simulink model "r2_b8a4x1kf"  (R2012b)
settings: Solver=VariableStepDiscrete  SolverMode=SingleTasking  StartTime=0.0  StopTime=1  RelTol=1e-3
undefined symbols (not defined in the file): fft_stages, n_bits_ants, n_bits_xengs
libraries: xbsIndex_r4 x22142, casper_library_misc x166, xbsReplacements_r4 x24, casper_library_delays x8, xps_library x5, casper_library_communications x4
(part 7 of 178)

== system r2_b8a4x1kf/bus_expand8 ==
  bus_in : Inport
  reinterpret1 : xbsIndex_r4/Reinterpret  force_arith_type=on  arith_type=Unsigned  force_bin_pt=on  bin_pt=0  block_type=reinterpret
  reinterpret2 : xbsIndex_r4/Reinterpret  force_arith_type=on  arith_type=Unsigned  force_bin_pt=on  bin_pt=0  block_type=reinterpret
  slice1 : xbsIndex_r4/Slice  nbits=16  boolean_output=off  mode=Upper Bit Location + Width  bit1=-16  base1=MSB of Input  bit0=0  base0=LSB of Input  dbl_ovrd=off  block_type=slice
  slice2 : xbsIndex_r4/Slice  nbits=16  boolean_output=off  mode=Upper Bit Location + Width  bit1=0  base1=MSB of Input  bit0=0  base0=LSB of Input  dbl_ovrd=off  block_type=slice
  msb_out2 : Outport
  lsb_out1 : Outport  Port=2
  wires:
  bus_in/1 -> slice2/1, slice1/1
  slice2/1 -> reinterpret2/1
  reinterpret2/1 -> msb_out2/1
  slice1/1 -> reinterpret1/1
  reinterpret1/1 -> lsb_out1/1

== system r2_b8a4x1kf/bus_expand9 ==
  bus_in : Inport
  slice1 : xbsIndex_r4/Slice  nbits=1  boolean_output=on  mode=Upper Bit Location + Width  bit1=-4  base1=MSB of Input  bit0=0  base0=LSB of Input  dbl_ovrd=off  block_type=slice
  slice2 : xbsIndex_r4/Slice  nbits=1  boolean_output=on  mode=Upper Bit Location + Width  bit1=-3  base1=MSB of Input  bit0=0  base0=LSB of Input  dbl_ovrd=off  block_type=slice
  slice3 : xbsIndex_r4/Slice  nbits=1  boolean_output=on  mode=Upper Bit Location + Width  bit1=-2  base1=MSB of Input  bit0=0  base0=LSB of Input  dbl_ovrd=off  block_type=slice
  slice4 : xbsIndex_r4/Slice  nbits=1  boolean_output=on  mode=Upper Bit Location + Width  bit1=-1  base1=MSB of Input  bit0=0  base0=LSB of Input  dbl_ovrd=off  block_type=slice
  slice5 : xbsIndex_r4/Slice  nbits=1  boolean_output=on  mode=Upper Bit Location + Width  bit1=0  base1=MSB of Input  bit0=0  base0=LSB of Input  dbl_ovrd=off  block_type=slice
  msb_out5 : Outport
  out4 : Outport  Port=2
  out3 : Outport  Port=3
  out2 : Outport  Port=4
  lsb_out1 : Outport  Port=5
  wires:
  bus_in/1 -> slice5/1, slice4/1, slice3/1, slice2/1, slice1/1
  slice5/1 -> msb_out5/1
  slice4/1 -> out4/1
  slice3/1 -> out3/1
  slice2/1 -> out2/1
  slice1/1 -> lsb_out1/1

== system r2_b8a4x1kf/control ==
  convert1_{1..8,10} (9 alike) : DataTypeConversion  OutDataTypeStr=fixdt('ufix1_En0')  LockScale=on
  convert1_9 : DataTypeConversion  OutDataTypeStr=fixdt('ufix2_En0')  LockScale=on
  convert2_{1..8,10} (9 alike) : DataTypeConversion  OutDataTypeStr=fixdt('ufix1_En0')  ConvertRealWorld=Stored Integer (SI)  LockScale=on
  convert2_9 : DataTypeConversion  OutDataTypeStr=fixdt('ufix2_En0')  ConvertRealWorld=Stored Integer (SI)  LockScale=on
  gain_1 : Gain  Gain=1024
  gain_10 : Gain
  gain_2 : Gain  Gain=512
  gain_3 : Gain  Gain=256
  gain_4 : Gain  Gain=128
  gain_5 : Gain  Gain=64
  gain_6 : Gain  Gain=32
  gain_7 : Gain  Gain=16
  gain_8 : Gain  Gain=8
  gain_9 : Gain  Gain=2
  io_delay : xbsIndex_r4/Delay  rst=off  infoeditControl=Selection of Reset will increase slice count due to use of real FFs and instead of SRLs  en=off  latency=0  dbl_ovrd=off  reg_retiming=on  block_type=delay
  r2_b8a4x1kf_new_control_user_data_out : xbsIndex_r4/Gateway In  gui_display_data_type=Fixed-point  arith_type=Unsigned  n_bits=32  bin_pt=0  preci_type=Single  exp_width=8  frac_width=24  quantization="Round  (unbiased: +/- Inf)"  overflow=Saturate  period=1  dbl_ovrd=off  timing_constraint=None  locs_specified=off  LOCs={}  UseAsADC=off  ADCChannel='1'  inherit_from_input=off  hdl_port=on  block_type=gatewayin
  reint9 : xbsIndex_r4/Reinterpret  force_arith_type=on  arith_type=Unsigned  force_bin_pt=on  bin_pt=0  block_type=reinterpret
  sim_{1..10} (10 alike) : Constant  Value=0
  sim_add : Sum  Inputs=++++++++++  OutDataTypeStr=uint32
  slice_cnt_rst : xbsIndex_r4/Slice  nbits=1  boolean_output=on  mode=Lower Bit Location + Width  bit1=0  base1=MSB of Input  bit0=8  base0=LSB of Input  dbl_ovrd=off  block_type=slice
  slice_flasher_en : xbsIndex_r4/Slice  nbits=1  boolean_output=on  mode=Lower Bit Location + Width  bit1=0  base1=MSB of Input  bit0=4  base0=LSB of Input  dbl_ovrd=off  block_type=slice
  slice_gbe_debug_rst : xbsIndex_r4/Slice  nbits=1  boolean_output=on  mode=Lower Bit Location + Width  bit1=0  base1=MSB of Input  bit0=5  base0=LSB of Input  dbl_ovrd=off  block_type=slice
  slice_gbe_rst : xbsIndex_r4/Slice  nbits=1  boolean_output=on  mode=Lower Bit Location + Width  bit1=0  base1=MSB of Input  bit0=7  base0=LSB of Input  dbl_ovrd=off  block_type=slice
  slice_gbe_txen : xbsIndex_r4/Slice  nbits=1  boolean_output=on  mode=Lower Bit Location + Width  bit1=0  base1=MSB of Input  bit0=6  base0=LSB of Input  dbl_ovrd=off  block_type=slice
  slice_reord_snaptrig : xbsIndex_r4/Slice  nbits=1  boolean_output=on  mode=Lower Bit Location + Width  bit1=0  base1=MSB of Input  bit0=3  base0=LSB of Input  dbl_ovrd=off  block_type=slice
  slice_reord_snaptrigsel : xbsIndex_r4/Slice  nbits=2  boolean_output=off  mode=Lower Bit Location + Width  bit1=0  base1=MSB of Input  bit0=1  base0=LSB of Input  dbl_ovrd=off  block_type=slice
  slice_status_clr : xbsIndex_r4/Slice  nbits=1  boolean_output=on  mode=Lower Bit Location + Width  bit1=0  base1=MSB of Input  bit0=9  base0=LSB of Input  dbl_ovrd=off  block_type=slice
  slice_unpack_snapwesel : xbsIndex_r4/Slice  nbits=1  boolean_output=on  mode=Lower Bit Location + Width  bit1=0  base1=MSB of Input  bit0=0  base0=LSB of Input  dbl_ovrd=off  block_type=slice
  slice_vacc_rst : xbsIndex_r4/Slice  nbits=1  boolean_output=on  mode=Lower Bit Location + Width  bit1=0  base1=MSB of Input  bit0=10  base0=LSB of Input  dbl_ovrd=off  block_type=slice
  in_vacc_rst : Outport
  in_status_clr : Outport  Port=2
  in_cnt_rst : Outport  Port=3
  in_gbe_rst : Outport  Port=4
  in_gbe_txen : Outport  Port=5
  in_gbe_debug_rst : Outport  Port=6
  in_flasher_en : Outport  Port=7
  in_reord_snaptrig : Outport  Port=8
  in_reord_snaptrigsel : Outport  Port=9
  in_unpack_snapwesel : Outport  Port=10
  wires:
  r2_b8a4x1kf_new_control_user_data_out/1 -> io_delay/1
  sim_add/1 -> r2_b8a4x1kf_new_control_user_data_out/1
  sim_1/1 -> convert1_1/1
  convert1_1/1 -> convert2_1/1
  convert2_1/1 -> gain_1/1
  gain_1/1 -> sim_add/1
  io_delay/1 -> slice_vacc_rst/1, slice_status_clr/1, slice_cnt_rst/1, slice_gbe_rst/1, slice_gbe_txen/1, slice_gbe_debug_rst/1, slice_flasher_en/1, slice_reord_snaptrig/1, slice_reord_snaptrigsel/1, slice_unpack_snapwesel/1
  slice_vacc_rst/1 -> in_vacc_rst/1
  sim_2/1 -> convert1_2/1
  convert1_2/1 -> convert2_2/1
  convert2_2/1 -> gain_2/1
  gain_2/1 -> sim_add/2
  slice_status_clr/1 -> in_status_clr/1
  sim_3/1 -> convert1_3/1
  convert1_3/1 -> convert2_3/1
  convert2_3/1 -> gain_3/1
  gain_3/1 -> sim_add/3
  slice_cnt_rst/1 -> in_cnt_rst/1
  sim_4/1 -> convert1_4/1
  convert1_4/1 -> convert2_4/1
  convert2_4/1 -> gain_4/1
  gain_4/1 -> sim_add/4
  slice_gbe_rst/1 -> in_gbe_rst/1
  sim_5/1 -> convert1_5/1
  convert1_5/1 -> convert2_5/1
  convert2_5/1 -> gain_5/1
  gain_5/1 -> sim_add/5
  slice_gbe_txen/1 -> in_gbe_txen/1
  sim_6/1 -> convert1_6/1
  convert1_6/1 -> convert2_6/1
  convert2_6/1 -> gain_6/1
  gain_6/1 -> sim_add/6
  slice_gbe_debug_rst/1 -> in_gbe_debug_rst/1
  sim_7/1 -> convert1_7/1
  convert1_7/1 -> convert2_7/1
  convert2_7/1 -> gain_7/1
  gain_7/1 -> sim_add/7
  slice_flasher_en/1 -> in_flasher_en/1
  sim_8/1 -> convert1_8/1
  convert1_8/1 -> convert2_8/1
  convert2_8/1 -> gain_8/1
  gain_8/1 -> sim_add/8
  slice_reord_snaptrig/1 -> in_reord_snaptrig/1
  sim_9/1 -> convert1_9/1
  convert1_9/1 -> convert2_9/1
  convert2_9/1 -> gain_9/1
  gain_9/1 -> sim_add/9
  slice_reord_snaptrigsel/1 -> reint9/1
  reint9/1 -> in_reord_snaptrigsel/1
  sim_10/1 -> convert1_10/1
  convert1_10/1 -> convert2_10/1
  convert2_10/1 -> gain_10/1
  gain_10/1 -> sim_add/10
  slice_unpack_snapwesel/1 -> in_unpack_snapwesel/1

== system r2_b8a4x1kf/dest_err_cnt0 ==
  out_reg : Inport
  assert_reg : xbsIndex_r4/Assert  assert_type=on  type_source=Explicitly  gui_display_data_type=Fixed-point  arith_type=Unsigned  n_bits=16  bin_pt=0  preci_type=Single  exp_width=8  frac_width=24  assert_rate=off  rate_source=Explicitly  period=1  output_port=on  block_type=assert
  cast_gw : xbsIndex_r4/Convert  gui_display_data_type=Fixed-point  arith_type=Unsigned  n_bits=32  bin_pt=0  float_type=Single  exp_bits=8  fraction_bits=24  quantization=Truncate  overflow=Wrap  en=off  latency=0  dbl_ovrd=off  pipeline=off  block_type=convert
  io_delay : xbsIndex_r4/Delay  rst=off  infoeditControl=Selection of Reset will increase slice count due to use of real FFs and instead of SRLs  en=off  latency=0  dbl_ovrd=off  reg_retiming=on  block_type=delay
  r2_b8a4x1kf_new_dest_err_cnt0_user_data_in : xbsIndex_r4/Gateway Out  inherit_from_input=off  hdl_port=on  timing_constraint=None  locs_specified=off  LOCs={}  UseAsDAC=off  DACChannel='1'  block_type=gatewayout
  reint1 : xbsIndex_r4/Reinterpret  force_arith_type=on  arith_type=Unsigned  force_bin_pt=on  bin_pt=0  block_type=reinterpret
  sim_out : Terminator
  wires:
  io_delay/1 -> cast_gw/1
  cast_gw/1 -> r2_b8a4x1kf_new_dest_err_cnt0_user_data_in/1
  r2_b8a4x1kf_new_dest_err_cnt0_user_data_in/1 -> sim_out/1
  out_reg/1 -> assert_reg/1
  assert_reg/1 -> reint1/1
  reint1/1 -> io_delay/1

== system r2_b8a4x1kf/dest_err_cnt1 ==
  out_reg : Inport
  assert_reg : xbsIndex_r4/Assert  assert_type=on  type_source=Explicitly  gui_display_data_type=Fixed-point  arith_type=Unsigned  n_bits=16  bin_pt=0  preci_type=Single  exp_width=8  frac_width=24  assert_rate=off  rate_source=Explicitly  period=1  output_port=on  block_type=assert
  cast_gw : xbsIndex_r4/Convert  gui_display_data_type=Fixed-point  arith_type=Unsigned  n_bits=32  bin_pt=0  float_type=Single  exp_bits=8  fraction_bits=24  quantization=Truncate  overflow=Wrap  en=off  latency=0  dbl_ovrd=off  pipeline=off  block_type=convert
  io_delay : xbsIndex_r4/Delay  rst=off  infoeditControl=Selection of Reset will increase slice count due to use of real FFs and instead of SRLs  en=off  latency=0  dbl_ovrd=off  reg_retiming=on  block_type=delay
  r2_b8a4x1kf_new_dest_err_cnt1_user_data_in : xbsIndex_r4/Gateway Out  inherit_from_input=off  hdl_port=on  timing_constraint=None  locs_specified=off  LOCs={}  UseAsDAC=off  DACChannel='1'  block_type=gatewayout
  reint1 : xbsIndex_r4/Reinterpret  force_arith_type=on  arith_type=Unsigned  force_bin_pt=on  bin_pt=0  block_type=reinterpret
  sim_out : Terminator
  wires:
  io_delay/1 -> cast_gw/1
  cast_gw/1 -> r2_b8a4x1kf_new_dest_err_cnt1_user_data_in/1
  r2_b8a4x1kf_new_dest_err_cnt1_user_data_in/1 -> sim_out/1
  out_reg/1 -> assert_reg/1
  assert_reg/1 -> reint1/1
  reint1/1 -> io_delay/1

== system r2_b8a4x1kf/dest_err_cnt2 ==
  out_reg : Inport
  assert_reg : xbsIndex_r4/Assert  assert_type=on  type_source=Explicitly  gui_display_data_type=Fixed-point  arith_type=Unsigned  n_bits=16  bin_pt=0  preci_type=Single  exp_width=8  frac_width=24  assert_rate=off  rate_source=Explicitly  period=1  output_port=on  block_type=assert
  cast_gw : xbsIndex_r4/Convert  gui_display_data_type=Fixed-point  arith_type=Unsigned  n_bits=32  bin_pt=0  float_type=Single  exp_bits=8  fraction_bits=24  quantization=Truncate  overflow=Wrap  en=off  latency=0  dbl_ovrd=off  pipeline=off  block_type=convert
  io_delay : xbsIndex_r4/Delay  rst=off  infoeditControl=Selection of Reset will increase slice count due to use of real FFs and instead of SRLs  en=off  latency=0  dbl_ovrd=off  reg_retiming=on  block_type=delay
  r2_b8a4x1kf_new_dest_err_cnt2_user_data_in : xbsIndex_r4/Gateway Out  inherit_from_input=off  hdl_port=on  timing_constraint=None  locs_specified=off  LOCs={}  UseAsDAC=off  DACChannel='1'  block_type=gatewayout
  reint1 : xbsIndex_r4/Reinterpret  force_arith_type=on  arith_type=Unsigned  force_bin_pt=on  bin_pt=0  block_type=reinterpret
  sim_out : Terminator
  wires:
  io_delay/1 -> cast_gw/1
  cast_gw/1 -> r2_b8a4x1kf_new_dest_err_cnt2_user_data_in/1
  r2_b8a4x1kf_new_dest_err_cnt2_user_data_in/1 -> sim_out/1
  out_reg/1 -> assert_reg/1
  assert_reg/1 -> reint1/1
  reint1/1 -> io_delay/1

== system r2_b8a4x1kf/dest_err_cnt3 ==
  out_reg : Inport
  assert_reg : xbsIndex_r4/Assert  assert_type=on  type_source=Explicitly  gui_display_data_type=Fixed-point  arith_type=Unsigned  n_bits=16  bin_pt=0  preci_type=Single  exp_width=8  frac_width=24  assert_rate=off  rate_source=Explicitly  period=1  output_port=on  block_type=assert
  cast_gw : xbsIndex_r4/Convert  gui_display_data_type=Fixed-point  arith_type=Unsigned  n_bits=32  bin_pt=0  float_type=Single  exp_bits=8  fraction_bits=24  quantization=Truncate  overflow=Wrap  en=off  latency=0  dbl_ovrd=off  pipeline=off  block_type=convert
  io_delay : xbsIndex_r4/Delay  rst=off  infoeditControl=Selection of Reset will increase slice count due to use of real FFs and instead of SRLs  en=off  latency=0  dbl_ovrd=off  reg_retiming=on  block_type=delay
  r2_b8a4x1kf_new_dest_err_cnt3_user_data_in : xbsIndex_r4/Gateway Out  inherit_from_input=off  hdl_port=on  timing_constraint=None  locs_specified=off  LOCs={}  UseAsDAC=off  DACChannel='1'  block_type=gatewayout
  reint1 : xbsIndex_r4/Reinterpret  force_arith_type=on  arith_type=Unsigned  force_bin_pt=on  bin_pt=0  block_type=reinterpret
  sim_out : Terminator
  wires:
  io_delay/1 -> cast_gw/1
  cast_gw/1 -> r2_b8a4x1kf_new_dest_err_cnt3_user_data_in/1
  r2_b8a4x1kf_new_dest_err_cnt3_user_data_in/1 -> sim_out/1
  out_reg/1 -> assert_reg/1
  assert_reg/1 -> reint1/1
  reint1/1 -> io_delay/1

== system r2_b8a4x1kf/edge_detect ==
  in : Inport
  Delay : xbsIndex_r4/Delay  rst=off  infoeditControl=Selection of Reset will increase slice count due to use of real FFs and instead of SRLs  en=off  latency=1  dbl_ovrd=off  reg_retiming=on  block_type=delay
      settings: xl_area=[0, 0, 0, 0, 0, 0, 0]
  Inverter : xbsIndex_r4/Inverter  en=off  latency=0  dbl_ovrd=off  block_type=inv
      settings: xl_area=[0, 0, 0, 0, 0, 0, 0]
  edge_op : xbsIndex_r4/Logical  logical_function=NOR  inputs=2  en=off  latency=0  precision=Full  arith_type=Unsigned  n_bits=8  bin_pt=2  align_bp=on  dbl_ovrd=off  block_type=logical
      settings: xl_area=[0, 0, 0, 0, 0, 0, 0]
  out : Outport
  wires:
  Inverter/1 -> edge_op/1
  edge_op/1 -> out/1
  in/1 -> Inverter/1, Delay/1
  Delay/1 -> edge_op/2

== system r2_b8a4x1kf/edge_detect1 ==
  in : Inport
  Delay : xbsIndex_r4/Delay  rst=off  infoeditControl=Selection of Reset will increase slice count due to use of real FFs and instead of SRLs  en=off  latency=1  dbl_ovrd=off  reg_retiming=on  block_type=delay
      settings: xl_area=[0, 0, 0, 0, 0, 0, 0]
  Inverter : xbsIndex_r4/Inverter  en=off  latency=0  dbl_ovrd=off  block_type=inv
      settings: xl_area=[0, 0, 0, 0, 0, 0, 0]
  edge_op : xbsIndex_r4/Logical  logical_function=NOR  inputs=2  en=off  latency=0  precision=Full  arith_type=Unsigned  n_bits=8  bin_pt=2  align_bp=on  dbl_ovrd=off  block_type=logical
      settings: xl_area=[0, 0, 0, 0, 0, 0, 0]
  out : Outport
  wires:
  Delay/1 -> edge_op/2
  in/1 -> Delay/1, Inverter/1
  edge_op/1 -> out/1
  Inverter/1 -> edge_op/1

== system r2_b8a4x1kf/edge_detect2 ==
  in : Inport
  Delay : xbsIndex_r4/Delay  rst=off  infoeditControl=Selection of Reset will increase slice count due to use of real FFs and instead of SRLs  en=off  latency=1  dbl_ovrd=off  reg_retiming=on  block_type=delay
      settings: xl_area=[0, 0, 0, 0, 0, 0, 0]
  Inverter : xbsIndex_r4/Inverter  en=off  latency=0  dbl_ovrd=off  block_type=inv
      settings: xl_area=[0, 0, 0, 0, 0, 0, 0]
  edge_op : xbsIndex_r4/Logical  logical_function=NOR  inputs=2  en=off  latency=0  precision=Full  arith_type=Unsigned  n_bits=8  bin_pt=2  align_bp=on  dbl_ovrd=off  block_type=logical
      settings: xl_area=[0, 0, 0, 0, 0, 0, 0]
  out : Outport
  wires:
  Delay/1 -> edge_op/2
  in/1 -> Delay/1, Inverter/1
  edge_op/1 -> out/1
  Inverter/1 -> edge_op/1

== system r2_b8a4x1kf/edge_detect3 ==
  in : Inport
  Delay : xbsIndex_r4/Delay  rst=off  infoeditControl=Selection of Reset will increase slice count due to use of real FFs and instead of SRLs  en=off  latency=1  dbl_ovrd=off  reg_retiming=on  block_type=delay
      settings: xl_area=[0, 0, 0, 0, 0, 0, 0]
  Inverter : xbsIndex_r4/Inverter  en=off  latency=0  dbl_ovrd=off  block_type=inv
      settings: xl_area=[0, 0, 0, 0, 0, 0, 0]
  edge_op : xbsIndex_r4/Logical  logical_function=NOR  inputs=2  en=off  latency=0  precision=Full  arith_type=Unsigned  n_bits=8  bin_pt=2  align_bp=on  dbl_ovrd=off  block_type=logical
      settings: xl_area=[0, 0, 0, 0, 0, 0, 0]
  out : Outport
  wires:
  Inverter/1 -> edge_op/1
  edge_op/1 -> out/1
  in/1 -> Inverter/1, Delay/1
  Delay/1 -> edge_op/2

== system r2_b8a4x1kf/edge_detect5 ==
  in : Inport
  Delay : xbsIndex_r4/Delay  rst=off  infoeditControl=Selection of Reset will increase slice count due to use of real FFs and instead of SRLs  en=off  latency=1  dbl_ovrd=off  reg_retiming=on  block_type=delay
      settings: xl_area=[0, 0, 0, 0, 0, 0, 0]
  Inverter : xbsIndex_r4/Inverter  en=off  latency=0  dbl_ovrd=off  block_type=inv
      settings: xl_area=[0, 0, 0, 0, 0, 0, 0]
  edge_op : xbsIndex_r4/Logical  logical_function=NOR  inputs=2  en=off  latency=0  precision=Full  arith_type=Unsigned  n_bits=8  bin_pt=2  align_bp=on  dbl_ovrd=off  block_type=logical
      settings: xl_area=[0, 0, 0, 0, 0, 0, 0]
  out : Outport
  wires:
  Inverter/1 -> edge_op/1
  edge_op/1 -> out/1
  in/1 -> Inverter/1, Delay/1
  Delay/1 -> edge_op/2

== system r2_b8a4x1kf/flags0 ==
  convert1_1 : DataTypeConversion  OutDataTypeStr=fixdt('ufix1_En0')  LockScale=on
  convert1_2 : DataTypeConversion  OutDataTypeStr=fixdt('ufix15_En0')  LockScale=on
  convert2_1 : DataTypeConversion  OutDataTypeStr=fixdt('ufix1_En0')  ConvertRealWorld=Stored Integer (SI)  LockScale=on
  convert2_2 : DataTypeConversion  OutDataTypeStr=fixdt('ufix15_En0')  ConvertRealWorld=Stored Integer (SI)  LockScale=on
  gain_1 : Gain  Gain=32768
  gain_2 : Gain
  io_delay : xbsIndex_r4/Delay  rst=off  infoeditControl=Selection of Reset will increase slice count due to use of real FFs and instead of SRLs  en=off  latency=0  dbl_ovrd=off  reg_retiming=on  block_type=delay
  r2_b8a4x1kf_new_flags0_user_data_out : xbsIndex_r4/Gateway In  gui_display_data_type=Fixed-point  arith_type=Unsigned  n_bits=32  bin_pt=0  preci_type=Single  exp_width=8  frac_width=24  quantization="Round  (unbiased: +/- Inf)"  overflow=Saturate  period=1  dbl_ovrd=off  timing_constraint=None  locs_specified=off  LOCs={}  UseAsADC=off  ADCChannel='1'  inherit_from_input=off  hdl_port=on  block_type=gatewayin
  reint1 : xbsIndex_r4/Reinterpret  force_arith_type=on  arith_type=Unsigned  force_bin_pt=on  bin_pt=0  block_type=reinterpret
  reint2 : xbsIndex_r4/Reinterpret  force_arith_type=on  arith_type=Unsigned  force_bin_pt=on  bin_pt=0  block_type=reinterpret
  sim_1 : Constant  Value=0
  sim_2 : Constant  Value=0
  sim_add : Sum  OutDataTypeStr=uint32
  slice_flags : xbsIndex_r4/Slice  nbits=15  boolean_output=off  mode=Lower Bit Location + Width  bit1=0  base1=MSB of Input  bit0=0  base0=LSB of Input  dbl_ovrd=off  block_type=slice
  slice_tvg_en : xbsIndex_r4/Slice  nbits=1  boolean_output=off  mode=Lower Bit Location + Width  bit1=0  base1=MSB of Input  bit0=15  base0=LSB of Input  dbl_ovrd=off  block_type=slice
  in_tvg_en : Outport
  in_flags : Outport  Port=2
  wires:
  r2_b8a4x1kf_new_flags0_user_data_out/1 -> io_delay/1
  sim_add/1 -> r2_b8a4x1kf_new_flags0_user_data_out/1
  sim_1/1 -> convert1_1/1
  convert1_1/1 -> convert2_1/1
  convert2_1/1 -> gain_1/1
  gain_1/1 -> sim_add/1
  io_delay/1 -> slice_tvg_en/1, slice_flags/1
  slice_tvg_en/1 -> reint1/1
  reint1/1 -> in_tvg_en/1
  sim_2/1 -> convert1_2/1
  convert1_2/1 -> convert2_2/1
  convert2_2/1 -> gain_2/1
  gain_2/1 -> sim_add/2
  slice_flags/1 -> reint2/1
  reint2/1 -> in_flags/1

== system r2_b8a4x1kf/flags1 ==
  convert1_1 : DataTypeConversion  OutDataTypeStr=fixdt('ufix1_En0')  LockScale=on
  convert1_2 : DataTypeConversion  OutDataTypeStr=fixdt('ufix15_En0')  LockScale=on
  convert2_1 : DataTypeConversion  OutDataTypeStr=fixdt('ufix1_En0')  ConvertRealWorld=Stored Integer (SI)  LockScale=on
  convert2_2 : DataTypeConversion  OutDataTypeStr=fixdt('ufix15_En0')  ConvertRealWorld=Stored Integer (SI)  LockScale=on
  gain_1 : Gain  Gain=32768
  gain_2 : Gain
  io_delay : xbsIndex_r4/Delay  rst=off  infoeditControl=Selection of Reset will increase slice count due to use of real FFs and instead of SRLs  en=off  latency=0  dbl_ovrd=off  reg_retiming=on  block_type=delay
  r2_b8a4x1kf_new_flags1_user_data_out : xbsIndex_r4/Gateway In  gui_display_data_type=Fixed-point  arith_type=Unsigned  n_bits=32  bin_pt=0  preci_type=Single  exp_width=8  frac_width=24  quantization="Round  (unbiased: +/- Inf)"  overflow=Saturate  period=1  dbl_ovrd=off  timing_constraint=None  locs_specified=off  LOCs={}  UseAsADC=off  ADCChannel='1'  inherit_from_input=off  hdl_port=on  block_type=gatewayin
  reint1 : xbsIndex_r4/Reinterpret  force_arith_type=on  arith_type=Unsigned  force_bin_pt=on  bin_pt=0  block_type=reinterpret
  reint2 : xbsIndex_r4/Reinterpret  force_arith_type=on  arith_type=Unsigned  force_bin_pt=on  bin_pt=0  block_type=reinterpret
  sim_1 : Constant  Value=0
  sim_2 : Constant  Value=0
  sim_add : Sum  OutDataTypeStr=uint32
  slice_flags : xbsIndex_r4/Slice  nbits=15  boolean_output=off  mode=Lower Bit Location + Width  bit1=0  base1=MSB of Input  bit0=0  base0=LSB of Input  dbl_ovrd=off  block_type=slice
  slice_tvg_en : xbsIndex_r4/Slice  nbits=1  boolean_output=off  mode=Lower Bit Location + Width  bit1=0  base1=MSB of Input  bit0=15  base0=LSB of Input  dbl_ovrd=off  block_type=slice
  in_tvg_en : Outport
  in_flags : Outport  Port=2
  wires:
  r2_b8a4x1kf_new_flags1_user_data_out/1 -> io_delay/1
  sim_add/1 -> r2_b8a4x1kf_new_flags1_user_data_out/1
  sim_1/1 -> convert1_1/1
  convert1_1/1 -> convert2_1/1
  convert2_1/1 -> gain_1/1
  gain_1/1 -> sim_add/1
  io_delay/1 -> slice_tvg_en/1, slice_flags/1
  slice_tvg_en/1 -> reint1/1
  reint1/1 -> in_tvg_en/1
  sim_2/1 -> convert1_2/1
  convert1_2/1 -> convert2_2/1
  convert2_2/1 -> gain_2/1
  gain_2/1 -> sim_add/2
  slice_flags/1 -> reint2/1
  reint2/1 -> in_flags/1

== system r2_b8a4x1kf/flags2 ==
  convert1_1 : DataTypeConversion  OutDataTypeStr=fixdt('ufix1_En0')  LockScale=on
  convert1_2 : DataTypeConversion  OutDataTypeStr=fixdt('ufix15_En0')  LockScale=on
  convert2_1 : DataTypeConversion  OutDataTypeStr=fixdt('ufix1_En0')  ConvertRealWorld=Stored Integer (SI)  LockScale=on
  convert2_2 : DataTypeConversion  OutDataTypeStr=fixdt('ufix15_En0')  ConvertRealWorld=Stored Integer (SI)  LockScale=on
  gain_1 : Gain  Gain=32768
  gain_2 : Gain
  io_delay : xbsIndex_r4/Delay  rst=off  infoeditControl=Selection of Reset will increase slice count due to use of real FFs and instead of SRLs  en=off  latency=0  dbl_ovrd=off  reg_retiming=on  block_type=delay
  r2_b8a4x1kf_new_flags2_user_data_out : xbsIndex_r4/Gateway In  gui_display_data_type=Fixed-point  arith_type=Unsigned  n_bits=32  bin_pt=0  preci_type=Single  exp_width=8  frac_width=24  quantization="Round  (unbiased: +/- Inf)"  overflow=Saturate  period=1  dbl_ovrd=off  timing_constraint=None  locs_specified=off  LOCs={}  UseAsADC=off  ADCChannel='1'  inherit_from_input=off  hdl_port=on  block_type=gatewayin
  reint1 : xbsIndex_r4/Reinterpret  force_arith_type=on  arith_type=Unsigned  force_bin_pt=on  bin_pt=0  block_type=reinterpret
  reint2 : xbsIndex_r4/Reinterpret  force_arith_type=on  arith_type=Unsigned  force_bin_pt=on  bin_pt=0  block_type=reinterpret
  sim_1 : Constant  Value=0
  sim_2 : Constant  Value=0
  sim_add : Sum  OutDataTypeStr=uint32
  slice_flags : xbsIndex_r4/Slice  nbits=15  boolean_output=off  mode=Lower Bit Location + Width  bit1=0  base1=MSB of Input  bit0=0  base0=LSB of Input  dbl_ovrd=off  block_type=slice
  slice_tvg_en : xbsIndex_r4/Slice  nbits=1  boolean_output=off  mode=Lower Bit Location + Width  bit1=0  base1=MSB of Input  bit0=15  base0=LSB of Input  dbl_ovrd=off  block_type=slice
  in_tvg_en : Outport
  in_flags : Outport  Port=2
  wires:
  r2_b8a4x1kf_new_flags2_user_data_out/1 -> io_delay/1
  sim_add/1 -> r2_b8a4x1kf_new_flags2_user_data_out/1
  sim_1/1 -> convert1_1/1
  convert1_1/1 -> convert2_1/1
  convert2_1/1 -> gain_1/1
  gain_1/1 -> sim_add/1
  io_delay/1 -> slice_tvg_en/1, slice_flags/1
  slice_tvg_en/1 -> reint1/1
  reint1/1 -> in_tvg_en/1
  sim_2/1 -> convert1_2/1
  convert1_2/1 -> convert2_2/1
  convert2_2/1 -> gain_2/1
  gain_2/1 -> sim_add/2
  slice_flags/1 -> reint2/1
  reint2/1 -> in_flags/1

== system r2_b8a4x1kf/flags3 ==
  convert1_1 : DataTypeConversion  OutDataTypeStr=fixdt('ufix1_En0')  LockScale=on
  convert1_2 : DataTypeConversion  OutDataTypeStr=fixdt('ufix15_En0')  LockScale=on
  convert2_1 : DataTypeConversion  OutDataTypeStr=fixdt('ufix1_En0')  ConvertRealWorld=Stored Integer (SI)  LockScale=on
  convert2_2 : DataTypeConversion  OutDataTypeStr=fixdt('ufix15_En0')  ConvertRealWorld=Stored Integer (SI)  LockScale=on
  gain_1 : Gain  Gain=32768
  gain_2 : Gain
  io_delay : xbsIndex_r4/Delay  rst=off  infoeditControl=Selection of Reset will increase slice count due to use of real FFs and instead of SRLs  en=off  latency=0  dbl_ovrd=off  reg_retiming=on  block_type=delay
  r2_b8a4x1kf_new_flags3_user_data_out : xbsIndex_r4/Gateway In  gui_display_data_type=Fixed-point  arith_type=Unsigned  n_bits=32  bin_pt=0  preci_type=Single  exp_width=8  frac_width=24  quantization="Round  (unbiased: +/- Inf)"  overflow=Saturate  period=1  dbl_ovrd=off  timing_constraint=None  locs_specified=off  LOCs={}  UseAsADC=off  ADCChannel='1'  inherit_from_input=off  hdl_port=on  block_type=gatewayin
  reint1 : xbsIndex_r4/Reinterpret  force_arith_type=on  arith_type=Unsigned  force_bin_pt=on  bin_pt=0  block_type=reinterpret
  reint2 : xbsIndex_r4/Reinterpret  force_arith_type=on  arith_type=Unsigned  force_bin_pt=on  bin_pt=0  block_type=reinterpret
  sim_1 : Constant  Value=0
  sim_2 : Constant  Value=0
  sim_add : Sum  OutDataTypeStr=uint32
  slice_flags : xbsIndex_r4/Slice  nbits=15  boolean_output=off  mode=Lower Bit Location + Width  bit1=0  base1=MSB of Input  bit0=0  base0=LSB of Input  dbl_ovrd=off  block_type=slice
  slice_tvg_en : xbsIndex_r4/Slice  nbits=1  boolean_output=off  mode=Lower Bit Location + Width  bit1=0  base1=MSB of Input  bit0=15  base0=LSB of Input  dbl_ovrd=off  block_type=slice
  in_tvg_en : Outport
  in_flags : Outport  Port=2
  wires:
  r2_b8a4x1kf_new_flags3_user_data_out/1 -> io_delay/1
  sim_add/1 -> r2_b8a4x1kf_new_flags3_user_data_out/1
  sim_1/1 -> convert1_1/1
  convert1_1/1 -> convert2_1/1
  convert2_1/1 -> gain_1/1
  gain_1/1 -> sim_add/1
  io_delay/1 -> slice_tvg_en/1, slice_flags/1
  slice_tvg_en/1 -> reint1/1
  reint1/1 -> in_tvg_en/1
  sim_2/1 -> convert1_2/1
  convert1_2/1 -> convert2_2/1
  convert2_2/1 -> gain_2/1
  gain_2/1 -> sim_add/2
  slice_flags/1 -> reint2/1
  reint2/1 -> in_flags/1

== system r2_b8a4x1kf/gapsize ==
  io_delay : xbsIndex_r4/Delay  rst=off  infoeditControl=Selection of Reset will increase slice count due to use of real FFs and instead of SRLs  en=off  latency=0  dbl_ovrd=off  reg_retiming=on  block_type=delay
  r2_b8a4x1kf_new_gapsize_user_data_out : xbsIndex_r4/Gateway In  gui_display_data_type=Fixed-point  arith_type=Unsigned  n_bits=32  bin_pt=0  preci_type=Single  exp_width=8  frac_width=24  quantization="Round  (unbiased: +/- Inf)"  overflow=Saturate  period=1  dbl_ovrd=off  timing_constraint=None  locs_specified=off  LOCs={}  UseAsADC=off  ADCChannel='1'  inherit_from_input=off  hdl_port=on  block_type=gatewayin
  reint1 : xbsIndex_r4/Reinterpret  force_arith_type=on  arith_type=Unsigned  force_bin_pt=on  bin_pt=0  block_type=reinterpret
  sim_1 : Constant  Value=0
  slice_gap_size : xbsIndex_r4/Slice  nbits=22  boolean_output=off  mode=Lower Bit Location + Width  bit1=0  base1=MSB of Input  bit0=0  base0=LSB of Input  dbl_ovrd=off  block_type=slice
  in_gap_size : Outport
  wires:
  r2_b8a4x1kf_new_gapsize_user_data_out/1 -> io_delay/1
  sim_1/1 -> r2_b8a4x1kf_new_gapsize_user_data_out/1
  io_delay/1 -> slice_gap_size/1
  slice_gap_size/1 -> reint1/1
  reint1/1 -> in_gap_size/1
